simulink model "QDrone_YOLO_Interrupt_Commander"  (R2021b)
settings: Solver=ode1  StartTime=0.0  StopTime=inf  FixedStep=0.001  RelTol=1e-3  EnableMultiTasking=on
InitFcn:
  | set_param(gcs, 'ZoomFactor','FitSystem')
model workspace (MAT data in the model file):
  target_system = 1
undefined symbols (not defined in the file): HIL, qc_get_step_size
libraries: quarc_library x49, simulink x23, simulink_extras x5
(part 1 of 3)
settings Model: SimulationMode=external  ExtModeTrigDuration=10000  Creator=dmadill  LastModifiedBy=user
settings SolverCC: AlgebraicLoopSolver=TrustRegion  PositivePriorityOrder=on
settings DataIOCC: LimitDataPoints=on  SaveFormat=Array  ReturnWorkspaceOutputs=off
settings DebuggingCC: SolverPrmCheckMsg=warning  SFUnexpectedBacktrackingDiag=warning  SFNoUnconditionalDefaultTransitionDiag=warning  SFExecutionAtInitializationDiag=none  SFMachineParentedDataDiag=warning  ArithmeticOperatorsInVariantConditions=warning
settings HardwareCC: ProdBitPerLong=64  ProdHWDeviceType=Intel->x86-64 (Linux 64)
settings ModelReferenceCC: PropagateSignalLabelsOutOfModel=off
settings SFSimCC: SimUseLocalCustomCode=off  CustomCodeUndefinedFunction=UseInterfaceOnly
settings RTWCC: Description=QUARC Linux x64 Target (QDrone) Using Toolchain  SystemTargetFile=quarc_linux_x64.tlc  TemplateMakefile=quarc_default_tmf  RTWUseLocalCustomCode=off  Toolchain=QUARC linux_x64 | gmake (64-bit Windows)  BuildConfiguration=Faster Runs
settings CodeAppCC: StateflowObjectComments=on
settings STFCustomTargetCC: ConcurrentExecutionCompliant=on  UseToolchainInfoCompliant=on  SystemTargetFile=quarc_linux_x64.tlc
settings GRTTargetCC: TargetLangStandard=C89/C90 (ANSI)  ParMdlRefBuildCompliant=off  CompOptLevelCompliant=off  CombineOutputUpdateFcns=off  MatFileLogging=off  CPPClassGenCompliant=off  GRTInterface=on  ExtMode=on  ExtModeMexFile=quarc_comm  ExtModeMexArgs='-w -d /tmp -uri %u -URI_Host tcpip://192.168.2.11:18001','tcpip://192.168.2.14:17001?retries=10'
settings ConfigComp: CovMetricSettings=dw  CovSaveCumulativeToWorkspaceVar=on  CovSaveSingleToWorkspaceVar=on  CovExternalEMLEnable=off  CovSFcnEnable=off

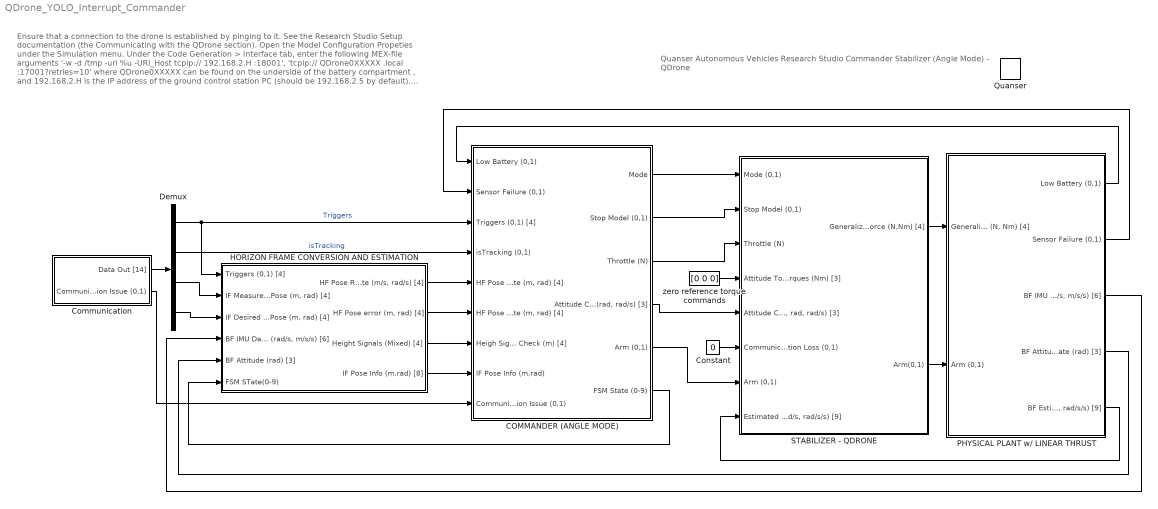
== system QDrone_YOLO_Interrupt_Commander ==
  note: Quanser Autonomous Vehicles Research Studio
      | Commander Stabilizer (Angle Mode) - QDrone
  note: Ensure that a connection to the drone is established by pinging to it. See the Research Studio Setup documentation (the Communicating with the QDrone section).
      | Open the Model Configuration Propeties under the Simulation menu.
      | Under the Code Generation > Interface tab, enter the following MEX-file arguments
      | '-w -d /tmp -uri %u -URI_Host tcpip:// 192.168.2.H :18001', 'tcpip:// QDrone0XXXXX .local :17001?retries=10'
      | where QDrone0XXXXX can be found on the underside of the battery compartment , and 192.168.2.H is the IP address of the ground control station PC (should be 192.168.2.5 by default).
      |
      | Under the QUARC menu, click on Build .
      |
      | Ensure that the associated Mission_Server model is running. If not, this model will stop immediately upon running. Click on Start under the QUARC menu.
      |
      | Ensure that the drone behaves as expected (see the steps in the associated Mission_Server model).
      | This model will automatically stop when the QDrone lands.
  COMMANDER (ANGLE MODE) : Subsystem
  Communication : Subsystem
  Constant : Constant  Value=0
  Demux : Demux  Outputs=[4 1 4 4]
  HORIZON FRAME CONVERSION AND ESTIMATION : Subsystem
  PHYSICAL PLANT w/ LINEAR THRUST : Subsystem
  Quanser : quarc_library/Logos/Quanser
  "STABILIZER - QDRONE " : Subsystem
  zero reference torque commands : Constant  Value=[0 0 0]
  wires:
  COMMANDER (ANGLE MODE)/2(Stop Model (0,1)) -> "STABILIZER - QDRONE "/2(Stop Model (0,1))
  zero reference torque commands/1 -> "STABILIZER - QDRONE "/4(Attitude Torques (Nm) [3])
  Communication/1(Data Out [14]) -> Demux/1
  PHYSICAL PLANT w/ LINEAR THRUST/1(Low Battery (0,1)) -> COMMANDER (ANGLE MODE)/1(Low Battery (0,1))
  PHYSICAL PLANT w/ LINEAR THRUST/2(Sensor Failure (0,1)) -> COMMANDER (ANGLE MODE)/2(Sensor Failure (0,1))
  Constant/1 -> "STABILIZER - QDRONE "/6(Communication Loss (0,1))
  COMMANDER (ANGLE MODE)/4("Attitude Commands (rad, rad/s) [3]") -> "STABILIZER - QDRONE "/5("Attitude Commands (rad, rad, rad/s) [3]")
  COMMANDER (ANGLE MODE)/1(Mode) -> "STABILIZER - QDRONE "/1(Mode (0,1))
  PHYSICAL PLANT w/ LINEAR THRUST/3("BF IMU Data (rad/s, m/s/s) [6]") -> HORIZON FRAME CONVERSION AND ESTIMATION/4("BF IMU Data (rad/s, m/s/s) [6]")
  Demux/3 -> HORIZON FRAME CONVERSION AND ESTIMATION/2("IF Measured Pose (m, rad) [4]")
  Demux/4 -> HORIZON FRAME CONVERSION AND ESTIMATION/3("IF Desired Pose (m, rad) [4]")
  Demux/1 -> COMMANDER (ANGLE MODE)/3(Triggers (0,1) [4]), HORIZON FRAME CONVERSION AND ESTIMATION/1(Triggers (0,1) [4])  "Triggers"
  Demux/2 -> COMMANDER (ANGLE MODE)/4(isTracking (0,1))  "isTracking"
  Communication/2(Communication Issue (0,1)) -> COMMANDER (ANGLE MODE)/9(Communication Issue (0,1))
  COMMANDER (ANGLE MODE)/6(FSM State (0-9)) -> HORIZON FRAME CONVERSION AND ESTIMATION/6(FSM STate(0-9))
  HORIZON FRAME CONVERSION AND ESTIMATION/1("HF Pose Rate Estimate (m/s, rad/s) [4]") -> COMMANDER (ANGLE MODE)/5("HF Pose Rate Estimate (m, rad) [4]")
  HORIZON FRAME CONVERSION AND ESTIMATION/2("HF Pose error (m, rad) [4]") -> COMMANDER (ANGLE MODE)/6("HF Pose Error Estimate (m, rad) [4]")
  HORIZON FRAME CONVERSION AND ESTIMATION/3(Height Signals (Mixed) [4]) -> COMMANDER (ANGLE MODE)/7(Heigh Signals Check (m) [4])
  HORIZON FRAME CONVERSION AND ESTIMATION/4(IF Pose Info (m,rad) [8]) -> COMMANDER (ANGLE MODE)/8(IF Pose Info (m,rad))
  COMMANDER (ANGLE MODE)/3(Throttle (N)) -> "STABILIZER - QDRONE "/3(Throttle (N))
  COMMANDER (ANGLE MODE)/5(Arm (0,1)) -> "STABILIZER - QDRONE "/7(Arm (0,1))
  PHYSICAL PLANT w/ LINEAR THRUST/5("BF Estimated Attitude (rad, rad/s, rad/s/s) [9]") -> "STABILIZER - QDRONE "/8("Estimated Attitude (rad, rad/s, rad/s/s) [9]")
  PHYSICAL PLANT w/ LINEAR THRUST/4(" BF Attitude Estimate (rad) [3]") -> HORIZON FRAME CONVERSION AND ESTIMATION/5(BF Attitude (rad) [3])
  "STABILIZER - QDRONE "/2(Arm(0,1)) -> PHYSICAL PLANT w/ LINEAR THRUST/2(Arm (0,1))
  "STABILIZER - QDRONE "/1(Generalized Force (N,Nm) [4]) -> PHYSICAL PLANT w/ LINEAR THRUST/1("Generalized Force (N, Nm) [4]")

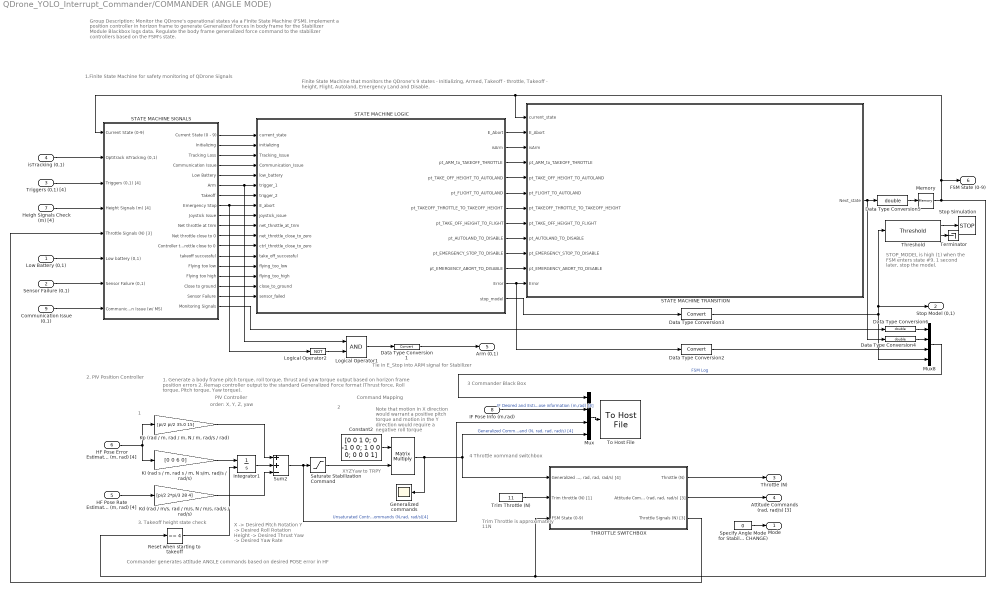
== system QDrone_YOLO_Interrupt_Commander/COMMANDER (ANGLE MODE) ==
  note: 1.Finite State Machine for safety monitoring of QDrone Signals
  note: 2. PIV Position Controller
  note: Commander generates attitude ANGLE commands based on desired POSE error in HF
  note: 3 Commander Black Box
  note: 4 Throttle xommand switchbox
  note: Group Description:
      |
      | Monitor the QDrone's operational states via a Finite State Machine (FSM).
      | Implement a position controller in horizon frame to generate Generalized Forces in body frame for the Stabilizer Module
      | Blackbox logs data.
      | Regulate the body frame generalized force command to the stabilizer controllers based on the FSM's state.
  note: Trim Throttle is approximately 11N
  note: Note that motion in X direction would warrant a positive pitch torque
      | and motion in the Y direction would require a negative roll torque
  note: Command Mapping
  note: XYZYaw to TRPY
  note: 1
  note: 3. Takeoff height state check
  note: order: X, Y, Z, yaw
  note: 1. Generate a body frame pitch torque, roll torque, thrust and yaw torque output based on horizon frame position errors
      | 2. Remap controller output to the standard Generalized Force format (Thrust force, Roll torque, Pitch torque, Yaw torque).
  note: 2
  note: PIV Controller
  note: X -> Desired Pitch Rotation
      | Y -> Desired Roll Rotation
      | Height -> Desired Thrust
      | Yaw -> Desired Yaw Rate
  note: Finite State Machine that monitors the QDrone's 9 states - Initializing, Armed, Takeoff - throttle, Takeoff - height, Flight, Autoland, Emergency Land and Disable.
  note: Tie in E_Stop into ARM signal for Stabilizer
  note: STOP_MODEL is high (1) when
      | the FSM enters state #9.
      | 1 second later, stop the model.
  Low Battery (0,1) : Inport
  Sensor Failure (0,1) : Inport  Port=2
  Triggers (0,1) [4] : Inport  Port=3
  isTracking (0,1) : Inport  Port=4
  "HF Pose Rate Estimate (m, rad) [4]" : Inport  Port=5
  "HF Pose Error Estimate (m, rad) [4]" : Inport  Port=6
  Heigh Signals Check (m) [4] : Inport  Port=7
  IF Pose Info (m,rad) : Inport  Port=8
  Communication Issue (0,1) : Inport  Port=9
  " " : Product  Multiplication=Matrix(*)
  Constant2 : Constant  Value=[0 0 1 0; 0 -1 0 0; 1 0 0 0; 0 0 0 1]
  Data Type Conversion1 : DataTypeConversion
  Data Type Conversion2 : DataTypeConversion
  Data Type Conversion3 : DataTypeConversion
  Data Type Conversion4 : DataTypeConversion  OutDataTypeStr=double
  Data Type Conversion5 : DataTypeConversion  OutDataTypeStr=double
  Data Type Conversion6 : DataTypeConversion  OutDataTypeStr=double
  "Generalized commands " : Scope
  Integrator1 : Integrator  ExternalReset=rising  LimitOutput=on  UpperSaturationLimit=[0.26 0.33 15 0.05].*0.75  LowerSaturationLimit=[-0.26 -0.33 -15 -0.05].*0.75
  "Kd (rad / m/s, rad / m/s, N / m/s, rad/s / rad/s)" : Gain  Gain=[pi/2 2*pi/3 28 4]
  "Ki (rad s / m, rad s / m, N s/m, rad/s / rad/s)" : Gain  Gain=[0 0 6 0]
  "Kp (rad / m, rad / m, N / m, rad/s / rad)" : Gain  Gain=[pi/2 pi/2 35.0 15]
  Logical Operator1 : Logic  AllPortsSameDT=off  OutDataTypeStr=boolean
  Logical Operator2 : Logic  Operator=NOT  AllPortsSameDT=off  OutDataTypeStr=boolean
  Memory : Memory  InitialCondition=1
  Mux : Mux
  Mux8 : Mux  Inputs=[17 1 1 1]
  Reset when starting to takeoff : simulink/Logic and Bit Operations/Compare To Constant  relop===  const=4  OutDataTypeStr=boolean
  STATE MACHINE LOGIC : MATLAB Function  TreatAsAtomicUnit=on
  STATE MACHINE SIGNALS : Subsystem
  STATE MACHINE TRANSITION : MATLAB Function  TreatAsAtomicUnit=on
  Saturate Stabilization Command : Saturate  UpperLimit=[pi/4 pi/4 35 100*pi/180]  LowerLimit=[-pi/4 -pi/4 -35 -100*pi/180]
  Specify Angle Mode for Stabilizer (DO NOT CHANGE) : Constant  Value=0
  Stop Simulation : Stop
  Sum2 : Sum  Inputs=++-
  "THROTTLE SWITCHBOX " : Subsystem
  Terminator : Terminator
  Threshold : quarc_library/Discontinuities/Threshold  operator=>=  param_src=Specify via dialog  threshold=0.5  duration=1
      settings: SourceProductName=QUARC Targets
  To Host File : quarc_library/Sinks/To Host/To Host File  file_name=saved_data/%m/Commander_%{date}_%{time}.mat  variable_name=commander_data  decimation=1  sample_time=-1  file_format=MAT-file v.5  options=No header or footer  append=off  final_file_name=saved_data/QDrone_YOLO_Interrupt_Commander/Commander_15-Sep-2026_10-49-51.mat  bitrate=2000000
  "Trim Throttle (N) " : Constant  Value=11
  Mode : Outport  VectorParamsAs1DForOutWhenUnconnected=off
  Stop Model (0,1) : Outport  Port=2  VectorParamsAs1DForOutWhenUnconnected=off
  Throttle (N) : Outport  Port=3  VectorParamsAs1DForOutWhenUnconnected=off
  "Attitude Commands (rad, rad/s) [3]" : Outport  Port=4  VectorParamsAs1DForOutWhenUnconnected=off
  Arm (0,1) : Outport  Port=5  VectorParamsAs1DForOutWhenUnconnected=off
  FSM State (0-9) : Outport  Port=6  VectorParamsAs1DForOutWhenUnconnected=off
  wires:
  Mux8/1 -> Mux/1  "FSM Log"
  Specify Angle Mode for Stabilizer (DO NOT CHANGE)/1 -> Mode/1
  "Trim Throttle (N) "/1 -> "THROTTLE SWITCHBOX "/2(Trim throttle (N) [1])
  "THROTTLE SWITCHBOX "/1(Throttle (N)) -> Throttle (N)/1
  "THROTTLE SWITCHBOX "/3(Throttle Signals (N) [3]) -> STATE MACHINE SIGNALS/5(Throttle Signals (N) [3])
  Mux/1 -> To Host File/1
  IF Pose Info (m,rad)/1 -> Mux/2  "IF Desired and Estimated  pose information (m,rad) [8]"
  "THROTTLE SWITCHBOX "/2("Attitude Command (rad, rad, rad/s) [3]") -> "Attitude Commands (rad, rad/s) [3]"/1
  Sum2/1 -> Mux/3, Saturate Stabilization Command/1  "Unsaturated Controller  Commands (N,rad, rad/s)[4]"
  "Ki (rad s / m, rad s / m, N s/m, rad/s / rad/s)"/1 -> Integrator1/1
  "Kd (rad / m/s, rad / m/s, N / m/s, rad/s / rad/s)"/1 -> Sum2/3
  "HF Pose Error Estimate (m, rad) [4]"/1 -> "Ki (rad s / m, rad s / m, N s/m, rad/s / rad/s)"/1, "Kp (rad / m, rad / m, N / m, rad/s / rad)"/1
  Saturate Stabilization Command/1 -> " "/2
  Constant2/1 -> " "/1
  Memory/1 -> Reset when starting to takeoff/1, "THROTTLE SWITCHBOX "/3(FSM State (0-9)), FSM State (0-9)/1, STATE MACHINE TRANSITION/1(current_state), STATE MACHINE SIGNALS/1(Current State (0-9))
  "HF Pose Rate Estimate (m, rad) [4]"/1 -> "Kd (rad / m/s, rad / m/s, N / m/s, rad/s / rad/s)"/1
  "Kp (rad / m, rad / m, N / m, rad/s / rad)"/1 -> Sum2/1
  Integrator1/1 -> Sum2/2
  Reset when starting to takeoff/1 -> Integrator1/2
  " "/1 -> "Generalized commands "/1, "THROTTLE SWITCHBOX "/1("Generalized Command (N, rad, rad, rad/s) [4]"), Mux/4  "Generalized Command (N, rad, rad, rad/s) [4]"
  STATE MACHINE SIGNALS/1("Current State (0 - 9)  ") -> STATE MACHINE LOGIC/1(current_state)
  Threshold/1 -> Stop Simulation/1
  STATE MACHINE LOGIC/3(pt_ARM_to_TAKEOFF_THROTTLE) -> STATE MACHINE TRANSITION/4(pt_ARM_to_TAKEOFF_THROTTLE)
  Data Type Conversion5/1 -> Memory/1
  STATE MACHINE SIGNALS/5(Low Battery) -> STATE MACHINE LOGIC/5(low_battery)
  STATE MACHINE SIGNALS/8(Emergency Stop) -> Logical Operator2/1, STATE MACHINE LOGIC/8(E_abort)
  Data Type Conversion6/1 -> Mux8/1
  STATE MACHINE SIGNALS/11(Net throttle close to 0) -> STATE MACHINE LOGIC/11(net_throttle_close_to_zero)
  STATE MACHINE SIGNALS/16(Close to ground) -> STATE MACHINE LOGIC/16(close_to_ground)
  STATE MACHINE LOGIC/6(pt_TAKEOFF_THROTTLE_TO_TAKEOFF_HEIGHT) -> STATE MACHINE TRANSITION/7(pt_TAKEOFF_THROTTLE_TO_TAKEOFF_HEIGHT)
  STATE MACHINE LOGIC/12(stop_model) -> Data Type Conversion3/1
  STATE MACHINE SIGNALS/13(takeoff successful) -> STATE MACHINE LOGIC/13(take_off_successful)
  STATE MACHINE SIGNALS/7(Takeoff) -> STATE MACHINE LOGIC/7(trigger_2)
  STATE MACHINE TRANSITION/1(Next_state) -> Data Type Conversion5/1, Data Type Conversion4/1
  STATE MACHINE SIGNALS/4(Communication Issue) -> STATE MACHINE LOGIC/4(Communication_Issue)
  STATE MACHINE LOGIC/9(pt_EMERGENCY_STOP_TO_DISABLE) -> STATE MACHINE TRANSITION/10(pt_EMERGENCY_STOP_TO_DISABLE)
  STATE MACHINE LOGIC/5(pt_FLIGHT_TO_AUTOLAND) -> STATE MACHINE TRANSITION/6(pt_FLIGHT_TO_AUTOLAND)
  STATE MACHINE LOGIC/1(E_Abort) -> STATE MACHINE TRANSITION/2(E_Abort)
  STATE MACHINE SIGNALS/9("Joystick Issue ") -> STATE MACHINE LOGIC/9(joystick_issue)
  Data Type Conversion4/1 -> Mux8/2
  STATE MACHINE SIGNALS/12(Controller throttle close to 0) -> STATE MACHINE LOGIC/12(ctrl_throttle_close_to_zero)
  STATE MACHINE SIGNALS/14(Flying too low) -> STATE MACHINE LOGIC/14(flying_too_low)
  STATE MACHINE SIGNALS/15(Flying too high) -> STATE MACHINE LOGIC/15(flying_too_high)
  STATE MACHINE SIGNALS/10(Net throttle at trim) -> STATE MACHINE LOGIC/10(net_throttle_at_trim)
  STATE MACHINE SIGNALS/3(Tracking Loss) -> STATE MACHINE LOGIC/3(Tracking_Issue)
  STATE MACHINE SIGNALS/2(Initializing) -> STATE MACHINE LOGIC/2(initializing)
  Data Type Conversion1/1 -> Arm (0,1)/1
  STATE MACHINE LOGIC/2(isArm) -> STATE MACHINE TRANSITION/3(isArm)
  Data Type Conversion3/1 -> Stop Model (0,1)/1, Threshold/1, Mux8/4
  STATE MACHINE LOGIC/4(pt_TAKE_OFF_HEIGHT_TO_AUTOLAND) -> STATE MACHINE TRANSITION/5(pt_TAKE_OFF_HEIGHT_TO_AUTOLAND)
  Threshold/2 -> Terminator/1
  Data Type Conversion2/1 -> Mux8/3
  Logical Operator1/1 -> Data Type Conversion1/1
  STATE MACHINE SIGNALS/6(Arm) -> Logical Operator1/1, STATE MACHINE LOGIC/6(trigger_1)
  STATE MACHINE SIGNALS/18(Monitoring Signals) -> Data Type Conversion6/1
  STATE MACHINE LOGIC/7(pt_TAKE_OFF_HEIGHT_TO_FLIGHT) -> STATE MACHINE TRANSITION/8(pt_TAKE_OFF_HEIGHT_TO_FLIGHT)
  Logical Operator2/1 -> Logical Operator1/2
  STATE MACHINE LOGIC/10(pt_EMERGENCY_ABORT_TO_DISABLE) -> STATE MACHINE TRANSITION/11(pt_EMERGENCY_ABORT_TO_DISABLE)
  STATE MACHINE LOGIC/8(pt_AUTOLAND_TO_DISABLE) -> STATE MACHINE TRANSITION/9(pt_AUTOLAND_TO_DISABLE)
  STATE MACHINE SIGNALS/17("  Sensor Failure") -> STATE MACHINE LOGIC/17(sensor_failed)
  STATE MACHINE LOGIC/11(Error) -> STATE MACHINE TRANSITION/12(Error), Data Type Conversion2/1
  Low Battery (0,1)/1 -> STATE MACHINE SIGNALS/6(Low battery (0,1))
  Sensor Failure (0,1)/1 -> STATE MACHINE SIGNALS/7(Sensor Failure (0,1))
  Communication Issue (0,1)/1 -> STATE MACHINE SIGNALS/8(Communication Issue (w/ MS))
  isTracking (0,1)/1 -> STATE MACHINE SIGNALS/2("Optitrack isTracking (0,1)  ")
  Triggers (0,1) [4]/1 -> STATE MACHINE SIGNALS/3(Triggers (0,1) [4])
  Heigh Signals Check (m) [4]/1 -> STATE MACHINE SIGNALS/4(Height Signals (m) [4])

== system QDrone_YOLO_Interrupt_Commander/Communication ==
  note: Argument (-URI_Host) is set at the MEX-file arguments found at Model Configuration Properties > Code Generation > Interface
      |
      | Format:
      | tcpip://192.168.2.H:18001
      | where H is the last digits of your ground station's IP address (use ipconfig in a command prompt to find it out).
  Constant : Constant
  Detect Communication Loss : Subsystem
  Memory : Memory  InheritSampleTime=on  LinearizeMemory=on  LinearizeAsDelay=on
  Model Argument : quarc_library/Sources/Signals/Model Argument  argument_name=URI_Host  has_value=on  data_type_mode=Specify via dialog  data_type=char  max_length=80  default_value=0  variable_size=off
      settings: AttributesFormatString=(-%<argument_name>)  SourceProductName=QUARC Targets
  Select Timestamp received and send back immediately (for calculating loopback time) : Selector  InputPortWidth=14  IndexOptions=Index vector (dialog)  Indices=[14]  OutputSizes=1
  Select the rest of the data : Selector  InputPortWidth=14  IndexOptions=Index vector (dialog)  Indices=[1:13]  OutputSizes=1
  Stream Client : quarc_library/Communications/Basic/Stream Client  uri_source=External input port  uri=tcpip://192.168.2.3:18669  send_buffer_size=1460  receive_buffer_size=1460  byte_order=little endian (Intel - LSB first)  optimization=Minimum latency  send_options=Send most recent data  receive_options=Receive most recent data  default_value=zeros(1,14)  sample_time=qc_get_step_size  active=off  implementation=Use blocking I/O in a separate thread  send_fifo_size=1000  receive_fifo_size=1000  send_priority=0  receive_priority=0  send_dimensions=off  receive_dimensions=off  max_dimensions=-1  data_type=Inherited via back propagation  type_expr=BusObject
  String Display : quarc_library/Strings/String Display  alignment=center  display_mode=Single line  sample_time=-1  use_new=off
      settings: SourceProductName=QUARC Targets
  Terminator1 : Terminator
  Terminator2 : Terminator
  Data Out [14] : Outport  VectorParamsAs1DForOutWhenUnconnected=off
  Communication Issue (0,1) : Outport  Port=2  VectorParamsAs1DForOutWhenUnconnected=off
  wires:
  Stream Client/5 -> Terminator2/1
  Model Argument/1 -> Stream Client/3, String Display/1
  Constant/1 -> Stream Client/2
  Stream Client/3 -> Terminator1/1
  Stream Client/4 -> Detect Communication Loss/3(Data Out), Select Timestamp received and send back immediately (for calculating loopback time)/1, Select the rest of the data/1
  Memory/1 -> Stream Client/1
  Stream Client/1 -> Detect Communication Loss/1(State)
  Stream Client/2 -> Detect Communication Loss/2(Error)
  Detect Communication Loss/1(Communication Issue) -> Communication Issue (0,1)/1
  Select the rest of the data/1 -> Data Out [14]/1  "isTracking Triggers IF Measured Pose  IF Desired Pose"
  Select Timestamp received and send back immediately (for calculating loopback time)/1 -> Memory/1

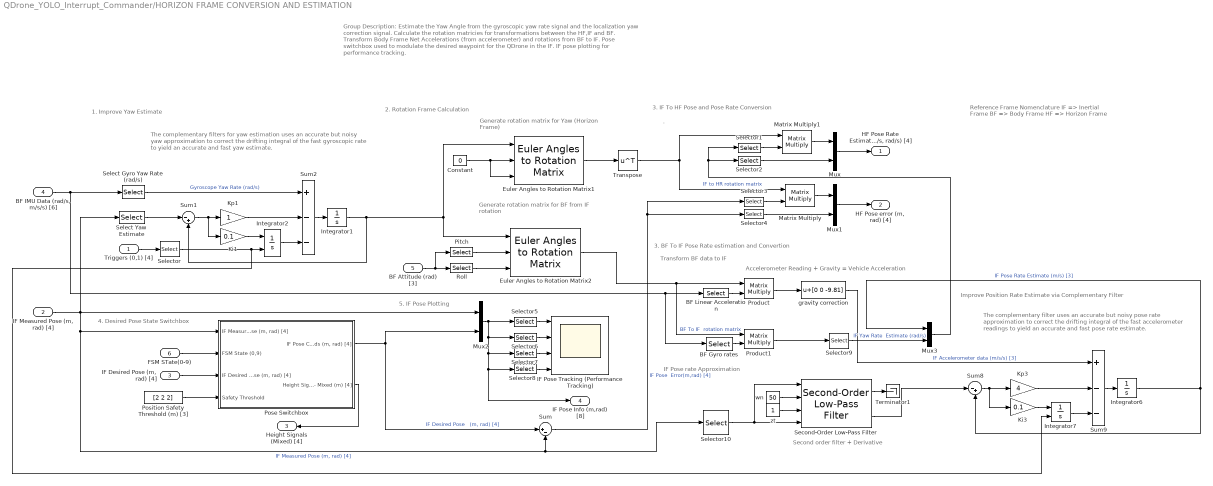
== system QDrone_YOLO_Interrupt_Commander/HORIZON FRAME CONVERSION AND ESTIMATION ==
  note: 3. IF To HF Pose and Pose Rate Conversion
  note: IF Pose rate Approximation
  note: Transform BF data to IF
  note: 3. BF To IF Pose Rate estimation and Convertion
  note: 2. Rotation Frame Calculation
  note: .
  note: Reference Frame Nomenclature
      | IF => Inertial Frame
      | BF => Body Frame
      | HF => Horizon Frame
  note: Group Description:
      |
      | Estimate the Yaw Angle from the gyroscopic yaw rate signal and the localization yaw correction signal.
      | Calculate the rotation matricies for transformations between the HF,IF and BF.
      | Transform Body Frame Net Accelerations (from accelerometer) and rotations from BF to IF.
      | Pose switchbox used to modulate the desired waypoint for the QDrone in the IF.
      | IF pose plotting for performance tracking.
  note: 4. Desired Pose State Switchbox
  note: 5. IF Pose Plotting
  note: 1. Improve Yaw Estimate
  note: The complementary filters for yaw estimation uses an accurate but noisy yaw approximation to correct the drifting integral of the fast gyroscopic rate to yield an accurate and fast yaw estimate.
  note: Generate rotation matrix for Yaw
      | (Horizon Frame)
  note: Generate rotation matrix
      | for BF from IF rotation
  note: Accelerometer Reading + Gravity = Vehicle Acceleration
  note: The complementary filter uses an accurate but noisy pose rate approximation to correct the drifting integral of the fast accelerometer readings to yield an accurate and fast pose rate estimate.
  note: Second order filter + Derivative
  note: Improve Position Rate Estimate via Complementary Filter
  Triggers (0,1) [4] : Inport
  "IF Measured Pose (m, rad) [4]" : Inport  Port=2
  "IF Desired Pose (m, rad) [4]" : Inport  Port=3
  "BF IMU Data (rad/s, m/s/s) [6]" : Inport  Port=4
  BF Attitude (rad) [3] : Inport  Port=5
  FSM STate(0-9) : Inport  Port=6
  BF Gyro rates : Selector  InputPortWidth=6  IndexOptions=Index vector (dialog)  Indices=[1:3]  OutputSizes=1
  BF Linear Acceleration : Selector  InputPortWidth=6  IndexOptions=Index vector (dialog)  Indices=[4:6]  OutputSizes=1
  Constant : Constant  Value=0
  Euler Angles to Rotation Matrix1 : quarc_library/Math Operations/Matrices/Euler Angles to Rotation Matrix  menu_order=Relative Z-Y-X
      settings: SourceProductName=QUARC Targets
  Euler Angles to Rotation Matrix2 : quarc_library/Math Operations/Matrices/Euler Angles to Rotation Matrix  menu_order=Relative Z-Y-X
      settings: SourceProductName=QUARC Targets
  IF Pose Tracking (Performance Tracking) : Scope  NumInputPorts=4
  Integrator1 : Integrator
  Integrator2 : Integrator  ExternalReset=rising
  Integrator6 : Integrator
  Integrator7 : Integrator  ExternalReset=rising
  Ki1 : Gain  Gain=0.1
  Ki3 : Gain  Gain=0.1
  Kp1 : Gain
  Kp3 : Gain  Gain=4
  Matrix Multiply : Product  Multiplication=Matrix(*)
  Matrix Multiply1 : Product  Multiplication=Matrix(*)
  Mux{,1..3} (4 alike) : Mux  Inputs=2
  Pitch : Selector  InputPortWidth=3  IndexOptions=Index vector (dialog)  Indices=[2]  OutputSizes=1
  Pose Switchbox : Subsystem
  Position Safety Threshold (m) [3] : Constant  Value=[2 2 2]
  Product : Product  Multiplication=Matrix(*)
  Product1 : Product  Multiplication=Matrix(*)
  Roll : Selector  InputPortWidth=3  IndexOptions=Index vector (dialog)  Indices=[1]  OutputSizes=1
  Second-Order Low-Pass Filter : quarc_library/Continuous/Second-Order Low-Pass Filter  params_source=External (input ports)  input_width=1  input_zeta=1  input_init=0
  Select Gyro Yaw Rate (rad/s) : Selector  InputPortWidth=6  IndexOptions=Index vector (dialog)  Indices=[3]  OutputSizes=1
  Select Yaw Estimate : Selector  InputPortWidth=4  IndexOptions=Index vector (dialog)  Indices=4  OutputSizes=1
  Selector : Selector  InputPortWidth=4  IndexOptions=Index vector (dialog)  Indices=[2]  OutputSizes=1
  Selector1 : Selector  InputPortWidth=4  IndexOptions=Index vector (dialog)  Indices=[1:3]  OutputSizes=1
  Selector10 : Selector  InputPortWidth=4  IndexOptions=Index vector (dialog)  Indices=[1:3]  OutputSizes=1
  Selector2 : Selector  InputPortWidth=4  IndexOptions=Index vector (dialog)  Indices=[4]  OutputSizes=1
  Selector3 : Selector  InputPortWidth=4  IndexOptions=Index vector (dialog)  Indices=[1:3]  OutputSizes=1
  Selector4 : Selector  InputPortWidth=4  IndexOptions=Index vector (dialog)  Indices=[4]  OutputSizes=1
  Selector5 : Selector  InputPortWidth=8  IndexOptions=Index vector (dialog)  Indices=[1 5]  OutputSizes=1
  Selector6 : Selector  InputPortWidth=8  IndexOptions=Index vector (dialog)  Indices=[2 6]  OutputSizes=1
  Selector7 : Selector  InputPortWidth=8  IndexOptions=Index vector (dialog)  Indices=[3 7]  OutputSizes=1
  Selector8 : Selector  InputPortWidth=8  IndexOptions=Index vector (dialog)  Indices=[4 8]  OutputSizes=1
  Selector9 : Selector  InputPortWidth=3  IndexOptions=Index vector (dialog)  Indices=[3]  OutputSizes=1
  Sum : Sum  Inputs=|+-
  Sum1 : Sum  Inputs=|-+
  Sum2 : Sum  Inputs=+--
  Sum8 : Sum  Inputs=|-+
  Sum9 : Sum  Inputs=+--
  Terminator1 : Terminator
  Transpose : Math  Operator=transpose  SignedPower=on  SaturateOnIntegerOverflow=on
  gravity correction : Bias  Bias=[0 0 -9.81]
  wn : Constant  Value=50
  zt : Constant
  "HF Pose Rate Estimate (m/s, rad/s) [4]" : Outport  VectorParamsAs1DForOutWhenUnconnected=off
  "HF Pose error (m, rad) [4]" : Outport  Port=2  VectorParamsAs1DForOutWhenUnconnected=off
  Height Signals (Mixed) [4] : Outport  Port=3  VectorParamsAs1DForOutWhenUnconnected=off
  IF Pose Info (m,rad) [8] : Outport  Port=4  VectorParamsAs1DForOutWhenUnconnected=off
  wires:
  Selector5/1 -> IF Pose Tracking (Performance Tracking)/1
  Selector7/1 -> IF Pose Tracking (Performance Tracking)/3
  Mux2/1 -> Selector6/1, Selector7/1, Selector8/1, IF Pose Info (m,rad) [8]/1, Selector5/1
  Selector6/1 -> IF Pose Tracking (Performance Tracking)/2
  Selector8/1 -> IF Pose Tracking (Performance Tracking)/4
  Selector4/1 -> Mux1/2
  Matrix Multiply/1 -> Mux1/1
  Selector3/1 -> Matrix Multiply/2
  Pose Switchbox/2(Height Signals - Mixed (m) [4]) -> Height Signals (Mixed) [4]/1
  Mux/1 -> "HF Pose Rate Estimate (m/s, rad/s) [4]"/1
  Selector2/1 -> Mux/2
  Selector1/1 -> Matrix Multiply1/2
  Matrix Multiply1/1 -> Mux/1
  Transpose/1 -> Matrix Multiply/1, Matrix Multiply1/1  "IF to HR rotation matrix"
  Mux3/1 -> Selector1/1, Selector2/1
  Mux1/1 -> "HF Pose error (m, rad) [4]"/1
  Sum/1 -> Selector3/1, Selector4/1  "IF Pose  Error(m,rad) [4]"
  FSM STate(0-9)/1 -> Pose Switchbox/2(FSM State (0,9))
  Position Safety Threshold (m) [3]/1 -> Pose Switchbox/4(Safety Threshold)
  "BF IMU Data (rad/s, m/s/s) [6]"/1 -> Select Gyro Yaw Rate (rad/s)/1, BF Linear Acceleration/1, BF Gyro rates/1
  Select Gyro Yaw Rate (rad/s)/1 -> Sum2/1  "Gyroscope Yaw Rate (rad/s)"
  Triggers (0,1) [4]/1 -> Selector/1
  BF Attitude (rad) [3]/1 -> Pitch/1, Roll/1
  "IF Desired Pose (m, rad) [4]"/1 -> Pose Switchbox/3("IF Desired Pose (m, rad) [4]")
  BF Linear Acceleration/1 -> Product/2
  BF Gyro rates/1 -> Product1/2
  Integrator2/1 -> Sum2/3
  Select Yaw Estimate/1 -> Sum1/1
  Sum1/1 -> Ki1/1, Kp1/1
  Kp1/1 -> Sum2/2
  Sum2/1 -> Integrator1/1
  Ki1/1 -> Integrator2/1
  Roll/1 -> Euler Angles to Rotation Matrix2/3
  Pitch/1 -> Euler Angles to Rotation Matrix2/2
  Constant/1 -> Euler Angles to Rotation Matrix1/3, Euler Angles to Rotation Matrix1/2
  Integrator1/1 -> Sum1/2, Euler Angles to Rotation Matrix2/1, Euler Angles to Rotation Matrix1/1
  Euler Angles to Rotation Matrix1/1 -> Transpose/1
  Product1/1 -> Selector9/1
  Product/1 -> gravity correction/1
  Euler Angles to Rotation Matrix2/1 -> Product/1, Product1/1  "BF To IF  rotation matrix"
  Selector10/1 -> Second-Order Low-Pass Filter/1, Second-Order Low-Pass Filter/4
  Kp3/1 -> Sum9/2
  gravity correction/1 -> Sum9/1  "IF Accelerometer data (m/s/s) [3]"
  Second-Order Low-Pass Filter/2 -> Sum8/1
  Second-Order Low-Pass Filter/1 -> Terminator1/1
  zt/1 -> Second-Order Low-Pass Filter/3
  Ki3/1 -> Integrator7/1
  Sum8/1 -> Ki3/1, Kp3/1
  Integrator6/1 -> Sum8/2, Mux3/1  "IF Pose Rate Estimate (m/s) [3]"
  Sum9/1 -> Integrator6/1
  wn/1 -> Second-Order Low-Pass Filter/2
  Integrator7/1 -> Sum9/3
  Selector/1 -> Integrator2/2, Integrator7/2
  Selector9/1 -> Mux3/2  "IF Yaw Rate  Estimate (rad/s)"
  "IF Measured Pose (m, rad) [4]"/1 -> Select Yaw Estimate/1, Sum/2, Selector10/1, Pose Switchbox/1("IF Measured Pose (m, rad) [4]"), Mux2/1  "IF Measured Pose (m, rad) [4]"
  Pose Switchbox/1("IF Pose Commands (m, rad) [4]") -> Mux2/2, Sum/1  "IF Desired Pose   (m, rad) [4]"

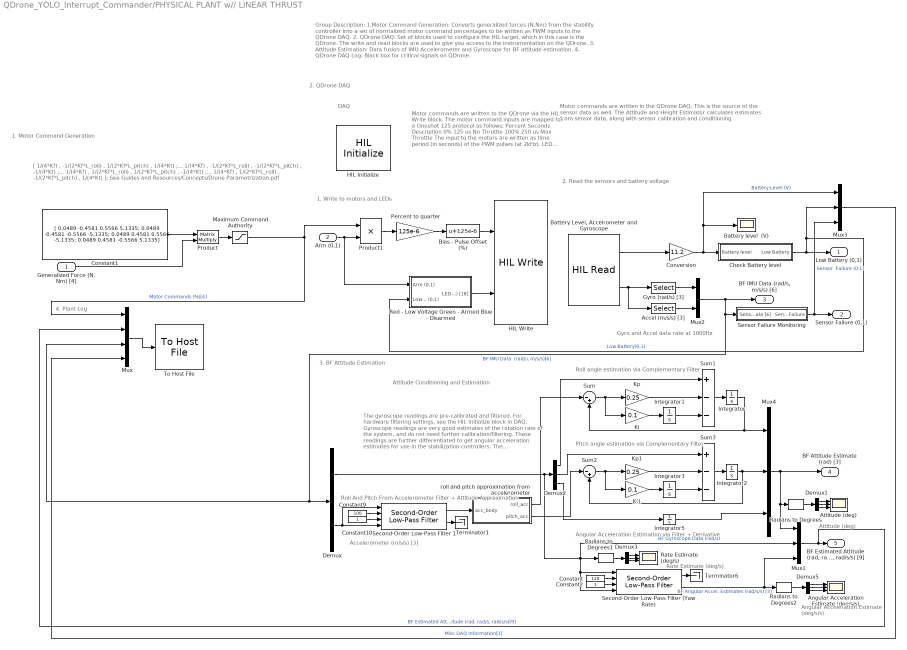
== system QDrone_YOLO_Interrupt_Commander/PHYSICAL PLANT w// LINEAR THRUST ==
  note: 3. BF Attitude Estimation
  note: 2. QDrone DAQ
  note: Group Description:
      |
      | 1.Motor Command Generation: Converts generalized forces (N,Nm) from the stability controller into a set of normalized motor command percentages to be written as PWM inputs to the QDrone DAQ.
      | 2. QDrone DAQ: Set of blocks used to configure the HIL target, which in this case is the QDrone. The write and read blocks are used to give you access to the instrumentation on the QDrone.
      | 3. Attitude Estimation: Data fusion of IMU Accelerometer and Gyroscope for BF attitude estimation.
      | 4. QDrone DAQ Log: Black box for critical signals on QDrone.
  note: 4. Plant Log
  note: [ 1/(4*Kf) , -1/(2*Kf*L_roll) , 1/(2*Kf*L_pitch) , 1/(4*Kt) ;...
      | 1/(4*Kf) , -1/(2*Kf*L_roll) , -1/(2*Kf*L_pitch) , -1/(4*Kt) ;...
      | 1/(4*Kf) , 1/(2*Kf*L_roll) , 1/(2*Kf*L_pitch) , -1/(4*Kt) ;...
      | 1/(4*Kf) , 1/(2*Kf*L_roll) , -1/(2*Kf*L_pitch) , 1/(4*Kt) ];
      |
      | See Guides and Resources/Concepts/Drone Parametrization.pdf
  note: Attitude (deg)
  note: Angular Acceleration
      | Estimate (deg/s/s)
  note: Motor commands are written in the QDrone DAQ. This is the source of the sensor data as well. The Attitude and Height Estimator calculates estimates from sensor data, along with sensor calibration and conditioning.
  note: 1. Motor Command Generation
  note: Gyro and Accel data rate at 1000Hz
  note: 2. Read the sensors and battery voltage
  note: 1. Write to motors and LEDs
  note: Motor commands are written to the QDrone via the HIL Write block. The motor command inputs are mapped for a Oneshot 125 protocol as follows:
      |
      | Percent Seconds Description
      | 0% 125 us No Throttle
      | 100% 250 us Max Throttle
      |
      | The input to the motors are written as time period (in seconds) of the PWM pulses (at 2kHz).
      |
      | LED colors can be set using a simple 3x1 ON (1) and OFF (0) vector (RGB mode).
  note: DAQ
  note: Angular Acceleration Estimation via Filter + Derivative
  note: The gyroscope readings are pre-calibrated and filtered. For hardware filtering settings, see the HIL Initialize block in DAQ. Gyroscope readings are very good estimates of the rotation rate of the system, and do not need further calibration/filtering. These readings are further differentiated to get angular acceleration estimates for use in the stabilization controllers.
      |
      | The accelerometer readings in body reference frame are used to calculate a roll and pitch approximation. This is based on the knowledge that the gravity vector points straight down.
  note: Roll angle estimation via Complementary Filter
  note: Pitch angle estimation via Complementary Filter
  note: Attitude Conditioning and Estimation
  note: Roll And Pitch From Accelerometer Filter + Attitude Approximation
  note: Accelerometer (m/s/s) [3]
  note: Rate Estimate (deg/s)
  "Generalized Force (N, Nm) [4]" : Inport
  Arm (0,1) : Inport  Port=2
  Accel (m/s/s) [3] : Selector  InputPortWidth=6  IndexOptions=Index vector (dialog)  Indices=[4:6]  OutputSizes=1
  Angular Acceleration Estimate (deg/s/s) : Scope  NumInputPorts=3
  Attitude (deg) : Scope  NumInputPorts=3
  "Battery Level, Accelrometer and Gyroscope" : quarc_library/Data Acquisition/Generic/Immediate I//O/HIL Read  Priority=1  object_name=HIL-1  analog_channels=[4]  encoder_channels=[]  digital_channels=[]  other_channels=[3000:3002 4000:4002]  sample_time=qc_get_step_size  active=on  vector_output=on  data_type_mode=Inherit via back propagation  encoder_data_type=double  digital_data_type=boolean
      settings: SourceProductName=The database C:\Users\user\AppData\Roaming\MathWorks\MATLAB\R2017a\slblocks_master.db is locked, or a table in the database is locked. (database is locked)
  Battery level  (V) : Scope
  Bias - Pulse Offset (%) : Bias  Bias=125e-6
  Check Battery level : Subsystem
  Constant : Constant  Value=120
  Constant1 : Constant  Value=|
      | [ 0.0489   -0.4581    0.5566    5.1335;
      |   0.0489   -0.4581   -0.5566   -5.1335;
      |   0.0489    0.4581    0.5566   -5.1335;
      |   0.0489    0.4581   -0.5566    5.1335]
  Constant10 : Constant
  Constant2 : Constant
  Constant9 : Constant  Value=100
  Conversion : Gain  Gain=11.2
  Demux : Demux  Outputs=[3 3]
  Demux{1..3,5} (4 alike) : Demux  Outputs=3
  Gyro (rad/s) [3] : Selector  InputPortWidth=6  IndexOptions=Index vector (dialog)  Indices=[1:3]  OutputSizes=1
  HIL Initialize : quarc_library/Data Acquisition/Generic/Configuration/HIL Initialize  object_name=HIL-1  board_type=qdrone  board_number=0  board_options=gyro_fs=2000;gyro_rate=1000;gyro_os=4;accel_fs=16;accel_rate=400;accel_os=4;baro_os=4096  exclusive=off  active=on  hardware_clocks=[]  clock_modes=[]  initial_clock_frequencies=[]  set_clock_params_at_start=off  set_clock_params_at_switch_in=off  set_clock_frequencies_at_start=off  set_clock_frequencies_at_switch_in=off  analog_input_channels=[0:4]  analog_input_configurations=[]  analog_input_maximums=[3.3]  analog_input_minimums=[0]  set_analog_input_params_at_start=off  set_analog_input_params_at_switch_in=off  analog_output_channels=[]  analog_output_maximums=[]  analog_output_minimums=[]  initial_analog_outputs=[]  final_analog_outputs=[]  watchdog_analog_outputs=[]  set_analog_output_params_at_start=off  set_analog_output_params_at_switch_in=off  set_analog_outputs_at_start=off  set_analog_outputs_at_switch_in=off  set_analog_outputs_at_terminate=off  set_analog_outputs_at_switch_out=off  set_analog_outputs_on_watchdog=off  digital_input_channels=[]  digital_output_channels=[5:7 9:23]  digital_output_configuration=[]  initial_digital_outputs=[0]  final_digital_outputs=[0]  watchdog_digital_outputs=[]  set_digital_output_params_at_start=off  set_digital_output_params_at_switch_in=off  set_digital_outputs_at_start=on  set_digital_outputs_at_switch_in=off  set_digital_outputs_at_terminate=on  set_digital_outputs_at_switch_out=off  set_digital_outputs_on_watchdog=off  encoder_channels=[0:2]  quadrature=[4]  encoder_filter_frequency=50e6/1  initial_encoder_counts=[0]  set_encoder_params_at_start=on  set_encoder_params_at_switch_in=off  set_encoder_counts_at_start=on  set_encoder_counts_at_switch_in=off  pwm_channels=[0:3]  pwm_modes=[4]  pwm_frequency=2000  pwm_configuration=[0]  pwm_alignment=[0]  pwm_polarity=[1]  pwm_leading_deadband=[]  pwm_trailing_deadband=[]  initial_pwm_outputs=[0]  final_pwm_outputs=[0]  watchdog_pwm_outputs=[0]  set_pwm_params_at_start=on  set_pwm_params_at_switch_in=off  set_pwm_outputs_at_start=on  set_pwm_outputs_at_switch_in=off  set_pwm_outputs_at_terminate=on  set_pwm_outputs_at_switch_out=off  set_pwm_outputs_on_watchdog=off  other_output_channels=[]  initial_other_outputs=[]  final_other_outputs=[]  watchdog_other_outputs=[]  set_other_outputs_at_start=off  set_other_outputs_at_switch_in=off  set_other_outputs_at_terminate=off  set_other_outputs_at_switch_out=off  set_other_outputs_on_watchdog=off
      settings: SourceProductName=The database C:\Users\user\AppData\Roaming\MathWorks\MATLAB\R2017a\slblocks_master.db is locked, or a table in the database is locked. (database is locked)
  HIL Write : quarc_library/Data Acquisition/Generic/Immediate I//O/HIL Write  object_name=HIL-1  analog_channels=[]  pwm_channels=[0:3]  digital_channels=[5:7 9:23]  other_channels=[]  sample_time=-1  active=off  vector_input=on
      settings: SourceProductName=The database C:\Users\user\AppData\Roaming\MathWorks\MATLAB\R2017a\slblocks_master.db is locked, or a table in the database is locked. (database is locked)
  Integrator{,1..3,5} (5 alike) : Integrator
  Ki : Gain  Gain=0.1
  Ki1 : Gain  Gain=0.1
  Kp : Gain  Gain=0.25
  Kp1 : Gain  Gain=0.25
  "Maximum Command Authority " : Saturate  UpperLimit=[1 1 1 1]  LowerLimit=[0 0 0 0]
  Mux : Mux
  Mux1 : Mux  Inputs=3
  Mux2 : Mux  Inputs=2
  Mux3 : Mux  Inputs=3
  Mux4 : Mux  Inputs=3
  Percent to quarter : Gain  Gain=125e-6
  Product : Product  Multiplication=Matrix(*)
  Product1 : Product
  Radians to Degrees : simulink_extras/Transformations/Radians to Degrees
  Radians to Degrees1 : simulink_extras/Transformations/Radians to Degrees
  Radians to Degrees2 : simulink_extras/Transformations/Radians to Degrees
  Rate Estimate (deg/s) : Scope  NumInputPorts=3
  Red - Low Voltage Green - Armed Blue - Disarmed : Subsystem
  Second-Order Low-Pass Filter (Yaw Rate) : quarc_library/Continuous/Second-Order Low-Pass Filter  params_source=External (input ports)  input_width=200  input_zeta=1  input_init=0
      settings: SourceProductName=The database C:\Users\user\AppData\Roaming\MathWorks\MATLAB\R2017a\slblocks_master.db is locked, or a table in the database is locked. (database is locked)
  Second-Order Low-Pass Filter 1 : quarc_library/Continuous/Second-Order Low-Pass Filter  params_source=External (input ports)  input_width=50  input_zeta=1  input_init=0
      settings: SourceProductName=The database C:\Users\user\AppData\Roaming\MathWorks\MATLAB\R2017a\slblocks_master.db is locked, or a table in the database is locked. (database is locked)
  Sensor Failure Monitoring : Subsystem
  Sum : Sum  Inputs=|-+
  Sum1 : Sum  Inputs=+--
  Sum2 : Sum  Inputs=|-+
  Sum3 : Sum  Inputs=+--
  Terminator1 : Terminator
  Terminator6 : Terminator
  To Host File : quarc_library/Sinks/To Host/To Host File  file_name=saved_data/%m/QDrone_%{date}_%{time}.mat  variable_name=QDrone_data  decimation=1  sample_time=-1  file_format=MAT-file v.5  options=No header or footer  append=off  final_file_name=saved_data/QDrone_YOLO_Interrupt_Commander/QDrone_15-Sep-2026_10-49-52.mat  bitrate=2000000
      settings: SourceProductName=The database C:\Users\user\AppData\Roaming\MathWorks\MATLAB\R2017a\slblocks_master.db is locked, or a table in the database is locked. (database is locked)
  roll and pitch approximation from accelerometer : MATLAB Function  TreatAsAtomicUnit=on
  Low Battery (0,1) : Outport  VectorParamsAs1DForOutWhenUnconnected=off
  Sensor Failure (0,1) : Outport  Port=2  VectorParamsAs1DForOutWhenUnconnected=off
  "BF IMU Data (rad/s, m/s/s) [6]" : Outport  Port=3  VectorParamsAs1DForOutWhenUnconnected=off
  " BF Attitude Estimate (rad) [3]" : Outport  Port=4  VectorParamsAs1DForOutWhenUnconnected=off
  "BF Estimated Attitude (rad, rad/s, rad/s/s) [9]" : Outport  Port=5  VectorParamsAs1DForOutWhenUnconnected=off
  wires:
  Demux1/1 -> Attitude (deg)/1
  Demux1/2 -> Attitude (deg)/2
  Demux1/3 -> Attitude (deg)/3
  Demux5/1 -> Angular Acceleration Estimate (deg/s/s)/1
  Demux5/2 -> Angular Acceleration Estimate (deg/s/s)/2
  Demux5/3 -> Angular Acceleration Estimate (deg/s/s)/3
  Radians to Degrees/1 -> Demux1/1
  Radians to Degrees2/1 -> Demux5/1
  "Maximum Command Authority "/1 -> Mux/1, Product1/1  "Motor Commands (%)[4]"
  Conversion/1 -> Check Battery level/1(Battery level), Mux3/1, Battery level  (V)/1  "Battery Level (V)"
  Constant1/1 -> Product/1
  "Generalized Force (N, Nm) [4]"/1 -> Product/2
  Product/1 -> "Maximum Command Authority "/1
  Mux/1 -> To Host File/1
  Accel (m/s/s) [3]/1 -> Mux2/2
  Product1/1 -> Percent to quarter/1
  Red - Low Voltage Green - Armed Blue - Disarmed/1(LEDs (%) [18]) -> HIL Write/2
  Bias - Pulse Offset (%)/1 -> HIL Write/1
  Percent to quarter/1 -> Bias - Pulse Offset (%)/1
  "Battery Level, Accelrometer and Gyroscope"/2 -> Accel (m/s/s) [3]/1, Gyro (rad/s) [3]/1
  "Battery Level, Accelrometer and Gyroscope"/1 -> Conversion/1
  Gyro (rad/s) [3]/1 -> Mux2/1
  Sensor Failure Monitoring/1(Sensor Failure) -> Sensor Failure (0,1)/1, Mux3/3  "Sensor  Failure (0,1)"
  Mux2/1 -> Mux/3, Demux/1, Sensor Failure Monitoring/1(Sensor Data [6]), "BF IMU Data (rad/s, m/s/s) [6]"/1  "BF IMU Data  (rad/s, m/s/s)[6]"
  Demux2/2 -> Sum3/1
  Integrator3/1 -> Sum3/3
  Integrator2/1 -> Sum2/2, Mux4/2
  Integrator5/1 -> Mux4/3
  Ki/1 -> Integrator1/1
  Demux2/1 -> Sum1/1
  Constant/1 -> Second-Order Low-Pass Filter (Yaw Rate)/2
  Integrator/1 -> Sum/2, Mux4/1
  Kp1/1 -> Sum3/2
  Sum2/1 -> Kp1/1, Ki1/1
  Sum3/1 -> Integrator2/1
  Sum1/1 -> Integrator/1
  Integrator1/1 -> Sum1/3
  Ki1/1 -> Integrator3/1
  Mux4/1 -> Radians to Degrees/1, Mux1/1, " BF Attitude Estimate (rad) [3]"/1
  Constant9/1 -> Second-Order Low-Pass Filter 1/2
  Second-Order Low-Pass Filter (Yaw Rate)/1 -> Terminator6/1
  Second-Order Low-Pass Filter 1/1 -> roll and pitch approximation from accelerometer/1(acc_body)
  roll and pitch approximation from accelerometer/1(roll_acc) -> Sum/1
  Demux2/3 -> Integrator5/1
  Sum/1 -> Ki/1, Kp/1
  Constant2/1 -> Second-Order Low-Pass Filter (Yaw Rate)/3
  Demux/2 -> Second-Order Low-Pass Filter 1/1, Second-Order Low-Pass Filter 1/4
  Constant10/1 -> Second-Order Low-Pass Filter 1/3
  Kp/1 -> Sum1/2
  roll and pitch approximation from accelerometer/2(pitch_acc) -> Sum2/1
  Second-Order Low-Pass Filter 1/2 -> Terminator1/1
  Second-Order Low-Pass Filter (Yaw Rate)/2 -> Radians to Degrees2/1, Mux1/3  "BF Angular Accel. Estimates (rad/s/s) [3]"
  Demux3/3 -> Rate Estimate (deg/s)/3
  Demux/1 -> Mux1/2, Radians to Degrees1/1, Second-Order Low-Pass Filter (Yaw Rate)/4, Second-Order Low-Pass Filter (Yaw Rate)/1, Demux2/1  "BF Gyroscope Data (rad/s)"
  Radians to Degrees1/1 -> Demux3/1
  Demux3/2 -> Rate Estimate (deg/s)/2
  Demux3/1 -> Rate Estimate (deg/s)/1
  Mux1/1 -> Mux/2, "BF Estimated Attitude (rad, rad/s, rad/s/s) [9]"/1  "BF Estimated Attitude (rad, rad/s, rad/s/s)[9]"
  Arm (0,1)/1 -> Red - Low Voltage Green - Armed Blue - Disarmed/1(Arm (0,1)), Product1/2
  Check Battery level/1(Low Battery) -> Mux3/2, Red - Low Voltage Green - Armed Blue - Disarmed/2(Low Battery (0,1)), Low Battery (0,1)/1  "Low Battery(0,1)"
  Mux3/1 -> Mux/4  "Misc DAQ Information[3]"

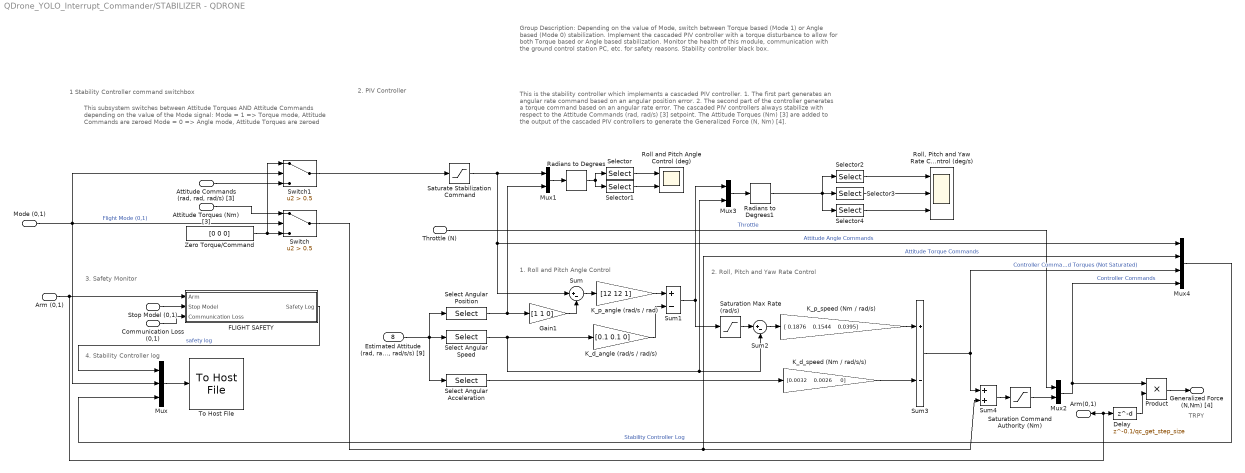
== system QDrone_YOLO_Interrupt_Commander/STABILIZER - QDRONE  ==
  note: 2. PIV Controller
  note: 4. Stability Controller log
  note: 1 Stability Controller command switchbox
  note: Group Description:
      |
      | Depending on the value of Mode, switch between Torque based (Mode 1) or Angle based (Mode 0) stabilization.
      | Implement the cascaded PIV controller with a torque disturbance to allow for both Torque based or Angle based stabilization.
      | Monitor the health of this module, communication with the ground control station PC, etc. for safety reasons.
      | Stability controller black box.
  note: TRPY
  note: 2. Roll, Pitch and Yaw Rate Control
  note: 1. Roll and Pitch Angle Control
  note: This is the stability controller which implements a cascaded PIV controller.
      | 1. The first part generates an angular rate command based on an angular position error.
      | 2. The second part of the controller generates a torque command based on an angular rate error.
      |
      | The cascaded PIV controllers always stabilize with respect to the Attitude Commands (rad, rad/s) [3] setpoint. The Attitude Torques (Nm) [3] are added to the output of the cascaded PIV controllers to generate the Generalized Force (N, Nm) [4].
  note: This subsystem switches between Attitude Torques AND Attitude Commands depending on
      | the value of the Mode signal:
      | Mode = 1	=> 		Torque mode, Attitude Commands are zeroed
      | Mode = 0	=> 		Angle mode, Attitude Torques are zeroed
  note: 3. Safety Monitor
  Mode (0,1) : Inport
  Stop Model (0,1) : Inport  Port=2
  Throttle (N) : Inport  Port=3
  Attitude Torques (Nm) [3] : Inport  Port=4
  "Attitude Commands (rad, rad, rad/s) [3]" : Inport  Port=5
  Communication Loss (0,1) : Inport  Port=6
  Arm (0,1) : Inport  Port=7
  "Estimated Attitude (rad, rad/s, rad/s/s) [9]" : Inport  Port=8
  Delay : Delay  DelayLength=0.1/qc_get_step_size
  FLIGHT SAFETY : Subsystem
  Gain1 : Gain  Gain=[1 1 0]
  K_d_angle (rad/s / rad/s) : Gain  Gain=[0.1 0.1 0]
  K_d_speed (Nm / rad/s/s) : Gain  Gain="[0.0032    0.0026     0]"
  K_p_angle (rad/s / rad) : Gain  Gain=[12 12 1]
  K_p_speed (Nm / rad/s) : Gain  Gain="[ 0.1876    0.1544    0.0395]"
  Mux : Mux  Inputs=3
  Mux1 : Mux  Inputs=2
  Mux2 : Mux  Inputs=2
  Mux3 : Mux  Inputs=2
  Mux4 : Mux
  Product : Product
  Radians to Degrees : simulink_extras/Transformations/Radians to Degrees
  Radians to Degrees1 : simulink_extras/Transformations/Radians to Degrees
  Roll and Pitch Angle Control (deg) : Scope  NumInputPorts=2
  "Roll, Pitch and Yaw Rate Control (deg/s)" : Scope  NumInputPorts=3
  Saturate Stabilization Command : Saturate  UpperLimit=[pi/4 pi/4 10*pi/18]  LowerLimit=[-pi/4 -pi/4 -10*pi/18]
  Saturation Command Authority (Nm) : Saturate  UpperLimit=[1.0915 0.8984 0.0984]  LowerLimit=-[1.0915 0.8984 0.0984]
  Saturation Max Rate (rad/s) : Saturate  UpperLimit=10*pi/3*[1 1 1]  LowerLimit=-10*pi/3*[1 1 1]
  Select Angular Acceleration : Selector  InputPortWidth=9  IndexOptions=Index vector (dialog)  Indices=[7:9]  OutputSizes=1
  Select Angular Speed : Selector  InputPortWidth=9  IndexOptions=Index vector (dialog)  Indices=[4:6]  OutputSizes=1
  Select Angular Position : Selector  InputPortWidth=9  IndexOptions=Index vector (dialog)  Indices=[1:3]  OutputSizes=1
  Selector : Selector  InputPortWidth=6  IndexOptions=Index vector (dialog)  Indices=[1 4]  OutputSizes=1
  Selector1 : Selector  InputPortWidth=6  IndexOptions=Index vector (dialog)  Indices=[2 5]  OutputSizes=1
  Selector2 : Selector  InputPortWidth=6  IndexOptions=Index vector (dialog)  Indices=[1 4]  OutputSizes=1
  Selector3 : Selector  InputPortWidth=6  IndexOptions=Index vector (dialog)  Indices=[2 5]  OutputSizes=1
  Selector4 : Selector  InputPortWidth=6  IndexOptions=Index vector (dialog)  Indices=[3 6]  OutputSizes=1
  Sum : Sum  Inputs=|+-
  Sum1 : Sum  Inputs=+-
  Sum2 : Sum  Inputs=|+-
  Sum3 : Sum  Inputs=+-
  Sum4 : Sum
  Switch : Switch  Criteria=u2 > Threshold  Threshold=0.5
  Switch1 : Switch  Criteria=u2 > Threshold  Threshold=0.5
  To Host File : quarc_library/Sinks/To Host/To Host File  file_name=saved_data/%m/Stabilizer_%{date}_%{time}.mat  variable_name=stabilizer_data  decimation=1  sample_time=-1  file_format=MAT-file v.5  options=No header or footer  append=off  final_file_name=saved_data/QDrone_YOLO_Interrupt_Commander/Stabilizer_15-Sep-2026_10-49-52.mat  bitrate=2000000
      settings: SourceProductName=The database C:\Users\user\AppData\Roaming\MathWorks\MATLAB\R2017a\slblocks_master.db is locked, or a table in the database is locked. (database is locked)
  Zero Torque/Command : Constant  Value=[0 0 0]
  Generalized Force (N,Nm) [4] : Outport  VectorParamsAs1DForOutWhenUnconnected=off
  Arm(0,1) : Outport  Port=2  VectorParamsAs1DForOutWhenUnconnected=off
  wires:
  Product/1 -> Generalized Force (N,Nm) [4]/1
  Stop Model (0,1)/1 -> FLIGHT SAFETY/2(Stop Model)
  Communication Loss (0,1)/1 -> FLIGHT SAFETY/3(Communication Loss)
  Mux/1 -> To Host File/1
  Mux4/1 -> Mux/3  "Stability Controller Log"
  Mode (0,1)/1 -> Switch/2, Switch1/2, Mux/2  "Flight Mode (0,1)"
  FLIGHT SAFETY/1(Safety Log) -> Mux/1  "safety log"
  K_p_speed (Nm / rad/s)/1 -> Sum3/1
  Sum/1 -> K_p_angle (rad/s / rad)/1
  K_d_speed (Nm / rad/s/s)/1 -> Sum3/2
  Arm (0,1)/1 -> Arm(0,1)/1, Delay/1, FLIGHT SAFETY/1(Arm)
  Mux3/1 -> Radians to Degrees1/1
  Sum1/1 -> Saturation Max Rate (rad/s)/1, Mux3/1
  Saturate Stabilization Command/1 -> Mux1/1, Sum/1, Mux4/1  "Attitude Angle Commands"
  Mux2/1 -> Mux4/4, Product/1  "Controller Commands"
  Select Angular Position/1 -> Mux1/2, Gain1/1
  Sum2/1 -> K_p_speed (Nm / rad/s)/1
  Throttle (N)/1 -> Mux2/1  "Throttle"
  Selector1/1 -> Roll and Pitch Angle Control (deg)/2
  Switch/1 -> Mux4/2, Sum4/2  "Attitude Torque Commands"
  Radians to Degrees1/1 -> Selector2/1, Selector4/1, Selector3/1
  "Estimated Attitude (rad, rad/s, rad/s/s) [9]"/1 -> Select Angular Position/1, Select Angular Acceleration/1, Select Angular Speed/1
  Mux1/1 -> Radians to Degrees/1
  Selector3/1 -> "Roll, Pitch and Yaw Rate Control (deg/s)"/2
  Sum4/1 -> Saturation Command Authority (Nm)/1
  Sum3/1 -> Mux4/3, Sum4/1  "Controller Command Torques (Not Saturated)"
  Saturation Command Authority (Nm)/1 -> Mux2/2
  Gain1/1 -> Sum/2
  Select Angular Acceleration/1 -> K_d_speed (Nm / rad/s/s)/1
  Switch1/1 -> Saturate Stabilization Command/1
  Saturation Max Rate (rad/s)/1 -> Sum2/1
  Selector4/1 -> "Roll, Pitch and Yaw Rate Control (deg/s)"/3
  K_p_angle (rad/s / rad)/1 -> Sum1/1
  Select Angular Speed/1 -> Sum2/2, Mux3/2, K_d_angle (rad/s / rad/s)/1
  Selector/1 -> Roll and Pitch Angle Control (deg)/1
  Selector2/1 -> "Roll, Pitch and Yaw Rate Control (deg/s)"/1
  K_d_angle (rad/s / rad/s)/1 -> Sum1/2
  Radians to Degrees/1 -> Selector/1, Selector1/1
  "Attitude Commands (rad, rad, rad/s) [3]"/1 -> Switch1/3
  Attitude Torques (Nm) [3]/1 -> Switch/1
  Zero Torque/Command/1 -> Switch1/1, Switch/3
  Delay/1 -> Product/2
